simulink model "s_c107m32k_vlbi"  (R2018a)
settings: Solver=VariableStepDiscrete  StartTime=0.0  StopTime=(2^15)*10  RelTol=1e-3
undefined symbols (not defined in the file): fft_stages, n_bits_xengs
libraries: xbsIndex_r4 x23049, casper_library_misc x45, xps_library x4, casper_library_scopes x3, simulink x2
(part 41 of 201)

== system s_c107m32k_vlbi/DDC/dec_fir_async2 ==
  sync_in : Inport
  dv_in : Inport  Port=2
  real1 : Inport  Port=3
  imag1 : Inport  Port=4
  real2 : Inport  Port=5
  imag2 : Inport  Port=6
  real3 : Inport  Port=7
  imag3 : Inport  Port=8
  real4 : Inport  Port=9
  imag4 : Inport  Port=10
  real5 : Inport  Port=11
  imag5 : Inport  Port=12
  real6 : Inport  Port=13
  imag6 : Inport  Port=14
  real7 : Inport  Port=15
  imag7 : Inport  Port=16
  real8 : Inport  Port=17
  imag8 : Inport  Port=18
  real9 : Inport  Port=19
  imag9 : Inport  Port=20
  real10 : Inport  Port=21
  imag10 : Inport  Port=22
  real11 : Inport  Port=23
  imag11 : Inport  Port=24
  real12 : Inport  Port=25
  imag12 : Inport  Port=26
  real13 : Inport  Port=27
  imag13 : Inport  Port=28
  real14 : Inport  Port=29
  imag14 : Inport  Port=30
  real15 : Inport  Port=31
  imag15 : Inport  Port=32
  real16 : Inport  Port=33
  imag16 : Inport  Port=34
  convert1 : Subsystem  AncestorBlock=casper_library_misc/convert_of  mask(convert_of){bit_width_i=43, binary_point_i=34, bit_width_o=18, binary_point_o=17, csp_latency=7, overflow=Saturate, quantization=Round  (unbiased: even values)}
      mask prompts: bit_width_i "Bit Width In"; binary_point_i "Binary Point In"; bit_width_o "Bit Width Out"; binary_point_o "Binary Point Out"; csp_latency "Latency"; overflow "Overflow Behaviour"; quantization "Quantization Behaviour"
      mask help:
      | Converts from one 2's complement bit-width
      | and/or binary point position to another.
      | Includes underflow/overflow indicator.
      mask init: same as s_c107m32k_vlbi/DDC/bus_convert/conv1
      settings: AttributesFormatString=[43,34]->[18,17]
      mask TypeOptions overflow: Wrap | Saturate | Error
      mask TypeOptions quantization: Truncate | Round  (unbiased: +/- Inf) | Round  (unbiased: even values)
  convert2 : Subsystem  AncestorBlock=casper_library_misc/convert_of  mask(convert_of){bit_width_i=43, binary_point_i=34, bit_width_o=18, binary_point_o=17, csp_latency=7, overflow=Saturate, quantization=Round  (unbiased: even values)}
      mask prompts: bit_width_i "Bit Width In"; binary_point_i "Binary Point In"; bit_width_o "Bit Width Out"; binary_point_o "Binary Point Out"; csp_latency "Latency"; overflow "Overflow Behaviour"; quantization "Quantization Behaviour"
      mask help:
      | Converts from one 2's complement bit-width
      | and/or binary point position to another.
      | Includes underflow/overflow indicator.
      mask init: same as s_c107m32k_vlbi/DDC/bus_convert/conv1
      settings: AttributesFormatString=[43,34]->[18,17]
      mask TypeOptions overflow: Wrap | Saturate | Error
      mask TypeOptions quantization: Truncate | Round  (unbiased: +/- Inf) | Round  (unbiased: even values)
  dv_delay : xbsIndex_r4/Delay  rst=off  infoeditControl=Selection of Reset will increase slice count due to use of real FFs and instead of SRLs  en=off  latency=8  reg_retiming=off  dbl_ovrd=off  block_type=delay
  fir_col_async1 : Subsystem  AncestorBlock=casper_library_downconverter/fir_col_async  mask(fir_col_async){n_inputs=16, coeff=[-0.00014496 -9.1553e-05 -4.5776e-05 -7.6294e-06  2.2888e-05  4.5776e-05  6.1035e-05  7.6294e-05  7.6294e-05  7.6294e-05  7.6294e-05  6.8665e-05  6.1035e-05  5.3406e-05  4.5776e-05  8.3923e-05], add_latency=7, mult_latency=7, coeff_bit_width=18, coeff_bin_pt=17, first_stage_hdl=on, adder_imp=DSP48, async=on, bus_input=off, input_width=0, input_bp=0, input_type=Signed, dbl=on}
      mask prompts: n_inputs "Inputs"; coeff "Coefficients"; add_latency "Add latency"; mult_latency "Mult Latency"; coeff_bit_width "Coefficient bit width"; coeff_bin_pt "Coefficient binary point"; first_stage_hdl "Implement first stage of adder trees on output as behavioural HDL"; adder_imp "Adder implementation"; async "Asynchronous ops"; bus_input "Bus input"; input_width "Input bitwidth"; input_bp "Input binary point"; input_type "Input datatype"; dbl "Double col"
      mask init:
      | fir_col_async_init(gcb);
      mask Help: eval('xlWeb(''http://casper.berkeley.edu/wiki/Fir_col'')')
      mask TypeOptions adder_imp: Behavioral | Fabric | DSP48
      mask Callback bus_input:
      | onoff = get_param(gcb, 'bus_input');
      | set_param_state(gcb, 'input_width', onoff)
      | set_param_state(gcb, 'input_bp', onoff)
      | set_param_state(gcb, 'input_type', onoff)
      mask TypeOptions input_type: Signed | Unsigned
  fir_col_async2 : Subsystem  AncestorBlock=casper_library_downconverter/fir_col_async  mask(fir_col_async){n_inputs=16, coeff=[-0.00064087 -0.00073242 -0.00079346  -0.0008316 -0.00084686 -0.00083923 -0.00080872 -0.00077057 -0.00071716  -0.0006485 -0.00057983 -0.00050354 -0.00042725 -0.00035095 -0.00027466 -0.00021362], add_latency=7, mult_latency=7, coeff_bit_width=18, coeff_bin_pt=17, first_stage_hdl=on, adder_imp=DSP48, async=on, bus_input=off, input_width=0, input_bp=0, input_type=Signed, dbl=on}
      mask prompts: n_inputs "Inputs"; coeff "Coefficients"; add_latency "Add latency"; mult_latency "Mult Latency"; coeff_bit_width "Coefficient bit width"; coeff_bin_pt "Coefficient binary point"; first_stage_hdl "Implement first stage of adder trees on output as behavioural HDL"; adder_imp "Adder implementation"; async "Asynchronous ops"; bus_input "Bus input"; input_width "Input bitwidth"; input_bp "Input binary point"; input_type "Input datatype"; dbl "Double col"
      mask init:
      | fir_col_async_init(gcb);
      mask Help: eval('xlWeb(''http://casper.berkeley.edu/wiki/Fir_col'')')
      mask TypeOptions adder_imp: Behavioral | Fabric | DSP48
      mask Callback bus_input:
      | onoff = get_param(gcb, 'bus_input');
      | set_param_state(gcb, 'input_width', onoff)
      | set_param_state(gcb, 'input_bp', onoff)
      | set_param_state(gcb, 'input_type', onoff)
      mask TypeOptions input_type: Signed | Unsigned
  fir_col_async3 : Subsystem  AncestorBlock=casper_library_downconverter/fir_col_async  mask(fir_col_async){n_inputs=16, coeff=[0.0018005   0.0018311   0.0018005   0.0017242   0.0016022    0.001442   0.0012589   0.0010529   0.0008316  0.00061035  0.00038147  0.00016785 -3.8147e-05 -0.00022125 -0.00038147 -0.00052643], add_latency=7, mult_latency=7, coeff_bit_width=18, coeff_bin_pt=17, first_stage_hdl=on, adder_imp=DSP48, async=on, bus_input=off, input_width=0, input_bp=0, input_type=Signed, dbl=on}
      mask prompts: n_inputs "Inputs"; coeff "Coefficients"; add_latency "Add latency"; mult_latency "Mult Latency"; coeff_bit_width "Coefficient bit width"; coeff_bin_pt "Coefficient binary point"; first_stage_hdl "Implement first stage of adder trees on output as behavioural HDL"; adder_imp "Adder implementation"; async "Asynchronous ops"; bus_input "Bus input"; input_width "Input bitwidth"; input_bp "Input binary point"; input_type "Input datatype"; dbl "Double col"
      mask init:
      | fir_col_async_init(gcb);
      mask Help: eval('xlWeb(''http://casper.berkeley.edu/wiki/Fir_col'')')
      mask TypeOptions adder_imp: Behavioral | Fabric | DSP48
      mask Callback bus_input:
      | onoff = get_param(gcb, 'bus_input');
      | set_param_state(gcb, 'input_width', onoff)
      | set_param_state(gcb, 'input_bp', onoff)
      | set_param_state(gcb, 'input_type', onoff)
      mask TypeOptions input_type: Signed | Unsigned
  fir_col_async4 : Subsystem  AncestorBlock=casper_library_downconverter/fir_col_async  mask(fir_col_async){n_inputs=16, coeff=[-0.0036469  -0.0034409  -0.0031433  -0.0027847  -0.0023651  -0.0019073  -0.0014343 -0.00094604 -0.00047302 -2.2888e-05  0.00039673  0.00077057   0.0010986   0.0013657   0.0015717   0.0017166], add_latency=7, mult_latency=7, coeff_bit_width=18, coeff_bin_pt=17, first_stage_hdl=on, adder_imp=DSP48, async=on, bus_input=off, input_width=0, input_bp=0, input_type=Signed, dbl=on}
      mask prompts: n_inputs "Inputs"; coeff "Coefficients"; add_latency "Add latency"; mult_latency "Mult Latency"; coeff_bit_width "Coefficient bit width"; coeff_bin_pt "Coefficient binary point"; first_stage_hdl "Implement first stage of adder trees on output as behavioural HDL"; adder_imp "Adder implementation"; async "Asynchronous ops"; bus_input "Bus input"; input_width "Input bitwidth"; input_bp "Input binary point"; input_type "Input datatype"; dbl "Double col"
      mask init:
      | fir_col_async_init(gcb);
      mask Help: eval('xlWeb(''http://casper.berkeley.edu/wiki/Fir_col'')')
      mask TypeOptions adder_imp: Behavioral | Fabric | DSP48
      mask Callback bus_input:
      | onoff = get_param(gcb, 'bus_input');
      | set_param_state(gcb, 'input_width', onoff)
      | set_param_state(gcb, 'input_bp', onoff)
      | set_param_state(gcb, 'input_type', onoff)
      mask TypeOptions input_type: Signed | Unsigned
  fir_col_async5 : Subsystem  AncestorBlock=casper_library_downconverter/fir_col_async  mask(fir_col_async){n_inputs=16, coeff=[0.005806    0.005043   0.0041809   0.0032578   0.0023041   0.0013504  0.00042725 -0.00045013  -0.0012512  -0.0019608  -0.0025635  -0.0030518  -0.0034103  -0.0036469  -0.0037613  -0.0037613], add_latency=7, mult_latency=7, coeff_bit_width=18, coeff_bin_pt=17, first_stage_hdl=on, adder_imp=DSP48, async=on, bus_input=off, input_width=0, input_bp=0, input_type=Signed, dbl=on}
      mask prompts: n_inputs "Inputs"; coeff "Coefficients"; add_latency "Add latency"; mult_latency "Mult Latency"; coeff_bit_width "Coefficient bit width"; coeff_bin_pt "Coefficient binary point"; first_stage_hdl "Implement first stage of adder trees on output as behavioural HDL"; adder_imp "Adder implementation"; async "Asynchronous ops"; bus_input "Bus input"; input_width "Input bitwidth"; input_bp "Input binary point"; input_type "Input datatype"; dbl "Double col"
      mask init:
      | fir_col_async_init(gcb);
      mask Help: eval('xlWeb(''http://casper.berkeley.edu/wiki/Fir_col'')')
      mask TypeOptions adder_imp: Behavioral | Fabric | DSP48
      mask Callback bus_input:
      | onoff = get_param(gcb, 'bus_input');
      | set_param_state(gcb, 'input_width', onoff)
      | set_param_state(gcb, 'input_bp', onoff)
      | set_param_state(gcb, 'input_type', onoff)
      mask TypeOptions input_type: Signed | Unsigned
  fir_col_async6 : Subsystem  AncestorBlock=casper_library_downconverter/fir_col_async  mask(fir_col_async){n_inputs=16, coeff=[-0.007637  -0.0057373  -0.0038147  -0.0019302 -0.00013733   0.0015335   0.0030365   0.0043335   0.0054169   0.0062637   0.0068665    0.007225   0.0073471   0.0072403   0.0069351   0.0064468], add_latency=7, mult_latency=7, coeff_bit_width=18, coeff_bin_pt=17, first_stage_hdl=on, adder_imp=DSP48, async=on, bus_input=off, input_width=0, input_bp=0, input_type=Signed, dbl=on}
      mask prompts: n_inputs "Inputs"; coeff "Coefficients"; add_latency "Add latency"; mult_latency "Mult Latency"; coeff_bit_width "Coefficient bit width"; coeff_bin_pt "Coefficient binary point"; first_stage_hdl "Implement first stage of adder trees on output as behavioural HDL"; adder_imp "Adder implementation"; async "Asynchronous ops"; bus_input "Bus input"; input_width "Input bitwidth"; input_bp "Input binary point"; input_type "Input datatype"; dbl "Double col"
      mask init:
      | fir_col_async_init(gcb);
      mask Help: eval('xlWeb(''http://casper.berkeley.edu/wiki/Fir_col'')')
      mask TypeOptions adder_imp: Behavioral | Fabric | DSP48
      mask Callback bus_input:
      | onoff = get_param(gcb, 'bus_input');
      | set_param_state(gcb, 'input_width', onoff)
      | set_param_state(gcb, 'input_bp', onoff)
      | set_param_state(gcb, 'input_type', onoff)
      mask TypeOptions input_type: Signed | Unsigned
  fir_col_async7 : Subsystem  AncestorBlock=casper_library_downconverter/fir_col_async  mask(fir_col_async){n_inputs=16, coeff=[0.0078812   0.0032501 -0.00092316  -0.0046005  -0.0077515   -0.010345   -0.012383   -0.013863   -0.014809   -0.015228   -0.015175   -0.014679   -0.013809   -0.012604   -0.011131  -0.0094528], add_latency=7, mult_latency=7, coeff_bit_width=18, coeff_bin_pt=17, first_stage_hdl=on, adder_imp=DSP48, async=on, bus_input=off, input_width=0, input_bp=0, input_type=Signed, dbl=on}
      mask prompts: n_inputs "Inputs"; coeff "Coefficients"; add_latency "Add latency"; mult_latency "Mult Latency"; coeff_bit_width "Coefficient bit width"; coeff_bin_pt "Coefficient binary point"; first_stage_hdl "Implement first stage of adder trees on output as behavioural HDL"; adder_imp "Adder implementation"; async "Asynchronous ops"; bus_input "Bus input"; input_width "Input bitwidth"; input_bp "Input binary point"; input_type "Input datatype"; dbl "Double col"
      mask init:
      | fir_col_async_init(gcb);
      mask Help: eval('xlWeb(''http://casper.berkeley.edu/wiki/Fir_col'')')
      mask TypeOptions adder_imp: Behavioral | Fabric | DSP48
      mask Callback bus_input:
      | onoff = get_param(gcb, 'bus_input');
      | set_param_state(gcb, 'input_width', onoff)
      | set_param_state(gcb, 'input_bp', onoff)
      | set_param_state(gcb, 'input_type', onoff)
      mask TypeOptions input_type: Signed | Unsigned
  fir_col_async8 : Subsystem  AncestorBlock=casper_library_downconverter/fir_col_async  mask(fir_col_async){n_inputs=16, coeff=[0.077705     0.07692    0.075363    0.073059    0.070053    0.066406    0.062187    0.057465     0.05233    0.046883    0.041206    0.035408    0.029587    0.023834    0.018242    0.012901], add_latency=7, mult_latency=7, coeff_bit_width=18, coeff_bin_pt=17, first_stage_hdl=on, adder_imp=DSP48, async=on, bus_input=off, input_width=0, input_bp=0, input_type=Signed, dbl=on}
      mask prompts: n_inputs "Inputs"; coeff "Coefficients"; add_latency "Add latency"; mult_latency "Mult Latency"; coeff_bit_width "Coefficient bit width"; coeff_bin_pt "Coefficient binary point"; first_stage_hdl "Implement first stage of adder trees on output as behavioural HDL"; adder_imp "Adder implementation"; async "Asynchronous ops"; bus_input "Bus input"; input_width "Input bitwidth"; input_bp "Input binary point"; input_type "Input datatype"; dbl "Double col"
      mask init:
      | fir_col_async_init(gcb);
      mask Help: eval('xlWeb(''http://casper.berkeley.edu/wiki/Fir_col'')')
      mask TypeOptions adder_imp: Behavioral | Fabric | DSP48
      mask Callback bus_input:
      | onoff = get_param(gcb, 'bus_input');
      | set_param_state(gcb, 'input_width', onoff)
      | set_param_state(gcb, 'input_bp', onoff)
      | set_param_state(gcb, 'input_type', onoff)
      mask TypeOptions input_type: Signed | Unsigned
  imag_sum : Subsystem  AncestorBlock=casper_library_misc/adder_tree  mask(adder_tree){n_inputs=8, csp_latency=7, adder_imp=DSP48, first_stage_hdl=off, floating_point=off, dvalid_en=on, float_type=single, frac_width=0, exp_width=0}
      mask prompts: n_inputs "Number of Inputs"; csp_latency "Add Latency"; adder_imp "Adder implementation"; first_stage_hdl "Use behavioural HDL for first stage of adders"; floating_point "floating point"; float_type "float type"; frac_width "fraction length"; exp_width "exponent length"
      mask help:
      | Sums all inputs using a tree of adds and delays.
      |
      | Number of inputs: The number of inputs to the block to be summed
      | Add latency: The number of clock cycles to perform one addition (affects timing)..
      | Adder implementation: choice of fabric or DSP48E core, or behavioral HDL
      | Use behavioural HDL for first stage of adders: Causes the first stage of adders to be absorbed into DSP blocks if multipliers precede them (Virtex 5). Overrides Adder implementation
      mask init: same as s_c107m32k_vlbi/DDC/dec_fir_async/imag_sum
      settings: AttributesFormatString=latency 21
      mask Help: eval('xlWeb(''http://casper.berkeley.edu/wiki/Adder_tree'')')
      mask TypeOptions adder_imp: Behavioral | Fabric | DSP48
      mask Callback floating_point:
      | onoff = get_param(gcb, 'floating_point');
      | if strcmp(onoff,'on')
      |     enable_fixpt = 'off'
      |     set_param_state(gcb, 'float_type', 'on')
      | 
      |     f_type = get_param(gcb, 'float_type')
      |     if strcmp(f_type,'custom')
      |         set_param_state(gcb, 'exp_width', 'on')
      |         set_param_state(gcb, 'frac_width', 'on')
      |     else
      |         set_param_state(gcb, 'exp_width', 'off')
      |         set_param_state(gcb, 'frac_width', 'off')
      |     end
      | 
      | 
      | else
      |     enable_fixpt = 'on'
      |     set_param_state(gcb, 'float_type', 'off')
      |     set_param_state(gcb, 'exp_width', 'off')
      |     set_param_state(gcb, 'frac_width', 'off')
      | end
      mask TypeOptions float_type: single | custom
      mask Callback float_type:
      | f_type = get_param(gcb, 'float_type')
      | if strcmp(f_type,'custom')
      |     set_param_state(gcb, 'exp_width', 'on')
      |     set_param_state(gcb, 'frac_width', 'on')
      | else
      |     set_param_state(gcb, 'exp_width', 'off')
      |     set_param_state(gcb, 'frac_width', 'off')
      | end
  or_reduce : xbsIndex_r4/Logical  logical_function=OR  inputs=2  en=off  latency=1  precision=Full  arith_type=Unsigned  n_bits=16  bin_pt=0  align_bp=on  dbl_ovrd=off  block_type=logical
  real_sum : Subsystem  AncestorBlock=casper_library_misc/adder_tree  mask(adder_tree){n_inputs=8, csp_latency=7, adder_imp=DSP48, first_stage_hdl=off, floating_point=off, dvalid_en=on, float_type=single, frac_width=0, exp_width=0}
      mask prompts: n_inputs "Number of Inputs"; csp_latency "Add Latency"; adder_imp "Adder implementation"; first_stage_hdl "Use behavioural HDL for first stage of adders"; floating_point "floating point"; float_type "float type"; frac_width "fraction length"; exp_width "exponent length"
      mask help:
      | Sums all inputs using a tree of adds and delays.
      |
      | Number of inputs: The number of inputs to the block to be summed
      | Add latency: The number of clock cycles to perform one addition (affects timing)..
      | Adder implementation: choice of fabric or DSP48E core, or behavioral HDL
      | Use behavioural HDL for first stage of adders: Causes the first stage of adders to be absorbed into DSP blocks if multipliers precede them (Virtex 5). Overrides Adder implementation
      mask init: same as s_c107m32k_vlbi/DDC/dec_fir_async/imag_sum
      settings: AttributesFormatString=latency 21
      mask Help: eval('xlWeb(''http://casper.berkeley.edu/wiki/Adder_tree'')')
      mask TypeOptions adder_imp: Behavioral | Fabric | DSP48
      mask Callback floating_point:
      | onoff = get_param(gcb, 'floating_point');
      | if strcmp(onoff,'on')
      |     enable_fixpt = 'off'
      |     set_param_state(gcb, 'float_type', 'on')
      | 
      |     f_type = get_param(gcb, 'float_type')
      |     if strcmp(f_type,'custom')
      |         set_param_state(gcb, 'exp_width', 'on')
      |         set_param_state(gcb, 'frac_width', 'on')
      |     else
      |         set_param_state(gcb, 'exp_width', 'off')
      |         set_param_state(gcb, 'frac_width', 'off')
      |     end
      | 
      | 
      | else
      |     enable_fixpt = 'on'
      |     set_param_state(gcb, 'float_type', 'off')
      |     set_param_state(gcb, 'exp_width', 'off')
      |     set_param_state(gcb, 'frac_width', 'off')
      | end
      mask TypeOptions float_type: single | custom
      mask Callback float_type:
      | f_type = get_param(gcb, 'float_type')
      | if strcmp(f_type,'custom')
      |     set_param_state(gcb, 'exp_width', 'on')
      |     set_param_state(gcb, 'frac_width', 'on')
      | else
      |     set_param_state(gcb, 'exp_width', 'off')
      |     set_param_state(gcb, 'frac_width', 'off')
      | end
  ri_to_c : casper_library_misc/ri_to_c
      settings: SourceProductName=CASPER DSP Blockset
  shift1 : xbsIndex_r4/Shift  shift_dir=Left  shift_bits=0  en=off  latency=1  precision=Full  arith_type="Signed  (2's comp)"  n_bits=16  bin_pt=14  quantization=Truncate  overflow=Wrap  dbl_ovrd=off  block_type=shift
  shift2 : xbsIndex_r4/Shift  shift_dir=Left  shift_bits=0  en=off  latency=1  precision=Full  arith_type="Signed  (2's comp)"  n_bits=16  bin_pt=14  quantization=Truncate  overflow=Wrap  dbl_ovrd=off  block_type=shift
  sync_delay : xbsIndex_r4/Delay  rst=off  infoeditControl=Selection of Reset will increase slice count due to use of real FFs and instead of SRLs  en=on  latency=49  reg_retiming=off  dbl_ovrd=off  block_type=delay
  sync_out : Outport
  dout : Outport  Port=2
  of_out : Outport  Port=3
  dv_out : Outport  Port=4
  wires:
  sync_in/1 -> sync_delay/1
  dv_in/1 -> dv_delay/1, sync_delay/2, fir_col_async1/65(dv), fir_col_async2/65(dv), fir_col_async3/65(dv), fir_col_async4/65(dv), fir_col_async5/65(dv), fir_col_async6/65(dv), fir_col_async7/65(dv), fir_col_async8/65(dv), real_sum/1(dv_in), imag_sum/1(dv_in)
  dv_delay/1 -> dv_out/1
  real1/1 -> fir_col_async1/1(real1)
  imag1/1 -> fir_col_async1/2(imag1)
  real2/1 -> fir_col_async1/3(real2)
  imag2/1 -> fir_col_async1/4(imag2)
  real3/1 -> fir_col_async1/5(real3)
  imag3/1 -> fir_col_async1/6(imag3)
  real4/1 -> fir_col_async1/7(real4)
  imag4/1 -> fir_col_async1/8(imag4)
  real5/1 -> fir_col_async1/9(real5)
  imag5/1 -> fir_col_async1/10(imag5)
  real6/1 -> fir_col_async1/11(real6)
  imag6/1 -> fir_col_async1/12(imag6)
  real7/1 -> fir_col_async1/13(real7)
  imag7/1 -> fir_col_async1/14(imag7)
  real8/1 -> fir_col_async1/15(real8)
  imag8/1 -> fir_col_async1/16(imag8)
  real9/1 -> fir_col_async1/17(real9)
  imag9/1 -> fir_col_async1/18(imag9)
  real10/1 -> fir_col_async1/19(real10)
  imag10/1 -> fir_col_async1/20(imag10)
  real11/1 -> fir_col_async1/21(real11)
  imag11/1 -> fir_col_async1/22(imag11)
  real12/1 -> fir_col_async1/23(real12)
  imag12/1 -> fir_col_async1/24(imag12)
  real13/1 -> fir_col_async1/25(real13)
  imag13/1 -> fir_col_async1/26(imag13)
  real14/1 -> fir_col_async1/27(real14)
  imag14/1 -> fir_col_async1/28(imag14)
  real15/1 -> fir_col_async1/29(real15)
  imag15/1 -> fir_col_async1/30(imag15)
  real16/1 -> fir_col_async1/31(real16)
  imag16/1 -> fir_col_async1/32(imag16)
  fir_col_async1/65(real_sum) -> real_sum/3(din1)
  fir_col_async1/66(imag_sum) -> imag_sum/3(din1)
  fir_col_async1/1(real_out1) -> fir_col_async2/1(real1)
  fir_col_async1/2(imag_out1) -> fir_col_async2/2(imag1)
  fir_col_async1/3(real_out2) -> fir_col_async2/3(real2)
  fir_col_async1/4(imag_out2) -> fir_col_async2/4(imag2)
  fir_col_async1/5(real_out3) -> fir_col_async2/5(real3)
  fir_col_async1/6(imag_out3) -> fir_col_async2/6(imag3)
  fir_col_async1/7(real_out4) -> fir_col_async2/7(real4)
  fir_col_async1/8(imag_out4) -> fir_col_async2/8(imag4)
  fir_col_async1/9(real_out5) -> fir_col_async2/9(real5)
  fir_col_async1/10(imag_out5) -> fir_col_async2/10(imag5)
  fir_col_async1/11(real_out6) -> fir_col_async2/11(real6)
  fir_col_async1/12(imag_out6) -> fir_col_async2/12(imag6)
  fir_col_async1/13(real_out7) -> fir_col_async2/13(real7)
  fir_col_async1/14(imag_out7) -> fir_col_async2/14(imag7)
  fir_col_async1/15(real_out8) -> fir_col_async2/15(real8)
  fir_col_async1/16(imag_out8) -> fir_col_async2/16(imag8)
  fir_col_async1/17(real_out9) -> fir_col_async2/17(real9)
  fir_col_async1/18(imag_out9) -> fir_col_async2/18(imag9)
  fir_col_async1/19(real_out10) -> fir_col_async2/19(real10)
  fir_col_async1/20(imag_out10) -> fir_col_async2/20(imag10)
  fir_col_async1/21(real_out11) -> fir_col_async2/21(real11)
  fir_col_async1/22(imag_out11) -> fir_col_async2/22(imag11)
  fir_col_async1/23(real_out12) -> fir_col_async2/23(real12)
  fir_col_async1/24(imag_out12) -> fir_col_async2/24(imag12)
  fir_col_async1/25(real_out13) -> fir_col_async2/25(real13)
  fir_col_async1/26(imag_out13) -> fir_col_async2/26(imag13)
  fir_col_async1/27(real_out14) -> fir_col_async2/27(real14)
  fir_col_async1/28(imag_out14) -> fir_col_async2/28(imag14)
  fir_col_async1/29(real_out15) -> fir_col_async2/29(real15)
  fir_col_async1/30(imag_out15) -> fir_col_async2/30(imag15)
  fir_col_async1/31(real_out16) -> fir_col_async2/31(real16)
  fir_col_async1/32(imag_out16) -> fir_col_async2/32(imag16)
  fir_col_async2/65(real_sum) -> real_sum/4(din2)
  fir_col_async2/66(imag_sum) -> imag_sum/4(din2)
  fir_col_async2/1(real_out1) -> fir_col_async3/1(real1)
  fir_col_async2/2(imag_out1) -> fir_col_async3/2(imag1)
  fir_col_async2/3(real_out2) -> fir_col_async3/3(real2)
  fir_col_async2/4(imag_out2) -> fir_col_async3/4(imag2)
  fir_col_async2/5(real_out3) -> fir_col_async3/5(real3)
  fir_col_async2/6(imag_out3) -> fir_col_async3/6(imag3)
  fir_col_async2/7(real_out4) -> fir_col_async3/7(real4)
  fir_col_async2/8(imag_out4) -> fir_col_async3/8(imag4)
  fir_col_async2/9(real_out5) -> fir_col_async3/9(real5)
  fir_col_async2/10(imag_out5) -> fir_col_async3/10(imag5)
  fir_col_async2/11(real_out6) -> fir_col_async3/11(real6)
  fir_col_async2/12(imag_out6) -> fir_col_async3/12(imag6)
  fir_col_async2/13(real_out7) -> fir_col_async3/13(real7)
  fir_col_async2/14(imag_out7) -> fir_col_async3/14(imag7)
  fir_col_async2/15(real_out8) -> fir_col_async3/15(real8)
  fir_col_async2/16(imag_out8) -> fir_col_async3/16(imag8)
  fir_col_async2/17(real_out9) -> fir_col_async3/17(real9)
  fir_col_async2/18(imag_out9) -> fir_col_async3/18(imag9)
  fir_col_async2/19(real_out10) -> fir_col_async3/19(real10)
  fir_col_async2/20(imag_out10) -> fir_col_async3/20(imag10)
  fir_col_async2/21(real_out11) -> fir_col_async3/21(real11)
  fir_col_async2/22(imag_out11) -> fir_col_async3/22(imag11)
  fir_col_async2/23(real_out12) -> fir_col_async3/23(real12)
  fir_col_async2/24(imag_out12) -> fir_col_async3/24(imag12)
  fir_col_async2/25(real_out13) -> fir_col_async3/25(real13)
  fir_col_async2/26(imag_out13) -> fir_col_async3/26(imag13)
  fir_col_async2/27(real_out14) -> fir_col_async3/27(real14)
  fir_col_async2/28(imag_out14) -> fir_col_async3/28(imag14)
  fir_col_async2/29(real_out15) -> fir_col_async3/29(real15)
  fir_col_async2/30(imag_out15) -> fir_col_async3/30(imag15)
  fir_col_async2/31(real_out16) -> fir_col_async3/31(real16)
  fir_col_async2/32(imag_out16) -> fir_col_async3/32(imag16)
  fir_col_async3/65(real_sum) -> real_sum/5(din3)
  fir_col_async3/66(imag_sum) -> imag_sum/5(din3)
  fir_col_async3/1(real_out1) -> fir_col_async4/1(real1)
  fir_col_async3/2(imag_out1) -> fir_col_async4/2(imag1)
  fir_col_async3/3(real_out2) -> fir_col_async4/3(real2)
  fir_col_async3/4(imag_out2) -> fir_col_async4/4(imag2)
  fir_col_async3/5(real_out3) -> fir_col_async4/5(real3)
  fir_col_async3/6(imag_out3) -> fir_col_async4/6(imag3)
  fir_col_async3/7(real_out4) -> fir_col_async4/7(real4)
  fir_col_async3/8(imag_out4) -> fir_col_async4/8(imag4)
  fir_col_async3/9(real_out5) -> fir_col_async4/9(real5)
  fir_col_async3/10(imag_out5) -> fir_col_async4/10(imag5)
  fir_col_async3/11(real_out6) -> fir_col_async4/11(real6)
  fir_col_async3/12(imag_out6) -> fir_col_async4/12(imag6)
  fir_col_async3/13(real_out7) -> fir_col_async4/13(real7)
  fir_col_async3/14(imag_out7) -> fir_col_async4/14(imag7)
  fir_col_async3/15(real_out8) -> fir_col_async4/15(real8)
  fir_col_async3/16(imag_out8) -> fir_col_async4/16(imag8)
  fir_col_async3/17(real_out9) -> fir_col_async4/17(real9)
  fir_col_async3/18(imag_out9) -> fir_col_async4/18(imag9)
  fir_col_async3/19(real_out10) -> fir_col_async4/19(real10)
  fir_col_async3/20(imag_out10) -> fir_col_async4/20(imag10)
  fir_col_async3/21(real_out11) -> fir_col_async4/21(real11)
  fir_col_async3/22(imag_out11) -> fir_col_async4/22(imag11)
  fir_col_async3/23(real_out12) -> fir_col_async4/23(real12)
  fir_col_async3/24(imag_out12) -> fir_col_async4/24(imag12)
  fir_col_async3/25(real_out13) -> fir_col_async4/25(real13)
  fir_col_async3/26(imag_out13) -> fir_col_async4/26(imag13)
  fir_col_async3/27(real_out14) -> fir_col_async4/27(real14)
  fir_col_async3/28(imag_out14) -> fir_col_async4/28(imag14)
  fir_col_async3/29(real_out15) -> fir_col_async4/29(real15)
  fir_col_async3/30(imag_out15) -> fir_col_async4/30(imag15)
  fir_col_async3/31(real_out16) -> fir_col_async4/31(real16)
  fir_col_async3/32(imag_out16) -> fir_col_async4/32(imag16)
  fir_col_async4/65(real_sum) -> real_sum/6(din4)
  fir_col_async4/66(imag_sum) -> imag_sum/6(din4)
  fir_col_async4/1(real_out1) -> fir_col_async5/1(real1)
  fir_col_async4/2(imag_out1) -> fir_col_async5/2(imag1)
  fir_col_async4/3(real_out2) -> fir_col_async5/3(real2)
  fir_col_async4/4(imag_out2) -> fir_col_async5/4(imag2)
  fir_col_async4/5(real_out3) -> fir_col_async5/5(real3)
  fir_col_async4/6(imag_out3) -> fir_col_async5/6(imag3)
  fir_col_async4/7(real_out4) -> fir_col_async5/7(real4)
  fir_col_async4/8(imag_out4) -> fir_col_async5/8(imag4)
  fir_col_async4/9(real_out5) -> fir_col_async5/9(real5)
  fir_col_async4/10(imag_out5) -> fir_col_async5/10(imag5)
  fir_col_async4/11(real_out6) -> fir_col_async5/11(real6)
  fir_col_async4/12(imag_out6) -> fir_col_async5/12(imag6)
  fir_col_async4/13(real_out7) -> fir_col_async5/13(real7)
  fir_col_async4/14(imag_out7) -> fir_col_async5/14(imag7)
  fir_col_async4/15(real_out8) -> fir_col_async5/15(real8)
  fir_col_async4/16(imag_out8) -> fir_col_async5/16(imag8)
  fir_col_async4/17(real_out9) -> fir_col_async5/17(real9)
  fir_col_async4/18(imag_out9) -> fir_col_async5/18(imag9)
  fir_col_async4/19(real_out10) -> fir_col_async5/19(real10)
  fir_col_async4/20(imag_out10) -> fir_col_async5/20(imag10)
  fir_col_async4/21(real_out11) -> fir_col_async5/21(real11)
  fir_col_async4/22(imag_out11) -> fir_col_async5/22(imag11)
  fir_col_async4/23(real_out12) -> fir_col_async5/23(real12)
  fir_col_async4/24(imag_out12) -> fir_col_async5/24(imag12)
  fir_col_async4/25(real_out13) -> fir_col_async5/25(real13)
  fir_col_async4/26(imag_out13) -> fir_col_async5/26(imag13)
  fir_col_async4/27(real_out14) -> fir_col_async5/27(real14)
  fir_col_async4/28(imag_out14) -> fir_col_async5/28(imag14)
  fir_col_async4/29(real_out15) -> fir_col_async5/29(real15)
  fir_col_async4/30(imag_out15) -> fir_col_async5/30(imag15)
  fir_col_async4/31(real_out16) -> fir_col_async5/31(real16)
  fir_col_async4/32(imag_out16) -> fir_col_async5/32(imag16)
  fir_col_async5/65(real_sum) -> real_sum/7(din5)
  fir_col_async5/66(imag_sum) -> imag_sum/7(din5)
  fir_col_async5/1(real_out1) -> fir_col_async6/1(real1)
  fir_col_async5/2(imag_out1) -> fir_col_async6/2(imag1)
  fir_col_async5/3(real_out2) -> fir_col_async6/3(real2)
  fir_col_async5/4(imag_out2) -> fir_col_async6/4(imag2)
  fir_col_async5/5(real_out3) -> fir_col_async6/5(real3)
  fir_col_async5/6(imag_out3) -> fir_col_async6/6(imag3)
  fir_col_async5/7(real_out4) -> fir_col_async6/7(real4)
  fir_col_async5/8(imag_out4) -> fir_col_async6/8(imag4)
  fir_col_async5/9(real_out5) -> fir_col_async6/9(real5)
  fir_col_async5/10(imag_out5) -> fir_col_async6/10(imag5)
  fir_col_async5/11(real_out6) -> fir_col_async6/11(real6)
  fir_col_async5/12(imag_out6) -> fir_col_async6/12(imag6)
  fir_col_async5/13(real_out7) -> fir_col_async6/13(real7)
  fir_col_async5/14(imag_out7) -> fir_col_async6/14(imag7)
  fir_col_async5/15(real_out8) -> fir_col_async6/15(real8)
  fir_col_async5/16(imag_out8) -> fir_col_async6/16(imag8)
  fir_col_async5/17(real_out9) -> fir_col_async6/17(real9)
  fir_col_async5/18(imag_out9) -> fir_col_async6/18(imag9)
  fir_col_async5/19(real_out10) -> fir_col_async6/19(real10)
  fir_col_async5/20(imag_out10) -> fir_col_async6/20(imag10)
  fir_col_async5/21(real_out11) -> fir_col_async6/21(real11)
  fir_col_async5/22(imag_out11) -> fir_col_async6/22(imag11)
  fir_col_async5/23(real_out12) -> fir_col_async6/23(real12)
  fir_col_async5/24(imag_out12) -> fir_col_async6/24(imag12)
  fir_col_async5/25(real_out13) -> fir_col_async6/25(real13)
  fir_col_async5/26(imag_out13) -> fir_col_async6/26(imag13)
  fir_col_async5/27(real_out14) -> fir_col_async6/27(real14)
  fir_col_async5/28(imag_out14) -> fir_col_async6/28(imag14)
  fir_col_async5/29(real_out15) -> fir_col_async6/29(real15)
  fir_col_async5/30(imag_out15) -> fir_col_async6/30(imag15)
  fir_col_async5/31(real_out16) -> fir_col_async6/31(real16)
  fir_col_async5/32(imag_out16) -> fir_col_async6/32(imag16)
  fir_col_async6/65(real_sum) -> real_sum/8(din6)
  fir_col_async6/66(imag_sum) -> imag_sum/8(din6)
  fir_col_async6/1(real_out1) -> fir_col_async7/1(real1)
  fir_col_async6/2(imag_out1) -> fir_col_async7/2(imag1)
  fir_col_async6/3(real_out2) -> fir_col_async7/3(real2)
  fir_col_async6/4(imag_out2) -> fir_col_async7/4(imag2)
  fir_col_async6/5(real_out3) -> fir_col_async7/5(real3)
  fir_col_async6/6(imag_out3) -> fir_col_async7/6(imag3)
  fir_col_async6/7(real_out4) -> fir_col_async7/7(real4)
  fir_col_async6/8(imag_out4) -> fir_col_async7/8(imag4)
  fir_col_async6/9(real_out5) -> fir_col_async7/9(real5)
  fir_col_async6/10(imag_out5) -> fir_col_async7/10(imag5)
  fir_col_async6/11(real_out6) -> fir_col_async7/11(real6)
  fir_col_async6/12(imag_out6) -> fir_col_async7/12(imag6)
  fir_col_async6/13(real_out7) -> fir_col_async7/13(real7)
  fir_col_async6/14(imag_out7) -> fir_col_async7/14(imag7)
  fir_col_async6/15(real_out8) -> fir_col_async7/15(real8)
  fir_col_async6/16(imag_out8) -> fir_col_async7/16(imag8)
  fir_col_async6/17(real_out9) -> fir_col_async7/17(real9)
  fir_col_async6/18(imag_out9) -> fir_col_async7/18(imag9)
  fir_col_async6/19(real_out10) -> fir_col_async7/19(real10)
  fir_col_async6/20(imag_out10) -> fir_col_async7/20(imag10)
  fir_col_async6/21(real_out11) -> fir_col_async7/21(real11)
  fir_col_async6/22(imag_out11) -> fir_col_async7/22(imag11)
  fir_col_async6/23(real_out12) -> fir_col_async7/23(real12)
  fir_col_async6/24(imag_out12) -> fir_col_async7/24(imag12)
  fir_col_async6/25(real_out13) -> fir_col_async7/25(real13)
  fir_col_async6/26(imag_out13) -> fir_col_async7/26(imag13)
  fir_col_async6/27(real_out14) -> fir_col_async7/27(real14)
  fir_col_async6/28(imag_out14) -> fir_col_async7/28(imag14)
  fir_col_async6/29(real_out15) -> fir_col_async7/29(real15)
  fir_col_async6/30(imag_out15) -> fir_col_async7/30(imag15)
  fir_col_async6/31(real_out16) -> fir_col_async7/31(real16)
  fir_col_async6/32(imag_out16) -> fir_col_async7/32(imag16)
  fir_col_async7/65(real_sum) -> real_sum/9(din7)
  fir_col_async7/66(imag_sum) -> imag_sum/9(din7)
  fir_col_async7/1(real_out1) -> fir_col_async8/1(real1)
  fir_col_async7/2(imag_out1) -> fir_col_async8/2(imag1)
  fir_col_async7/3(real_out2) -> fir_col_async8/3(real2)
  fir_col_async7/4(imag_out2) -> fir_col_async8/4(imag2)
  fir_col_async7/5(real_out3) -> fir_col_async8/5(real3)
  fir_col_async7/6(imag_out3) -> fir_col_async8/6(imag3)
  fir_col_async7/7(real_out4) -> fir_col_async8/7(real4)
  fir_col_async7/8(imag_out4) -> fir_col_async8/8(imag4)
  fir_col_async7/9(real_out5) -> fir_col_async8/9(real5)
  fir_col_async7/10(imag_out5) -> fir_col_async8/10(imag5)
  fir_col_async7/11(real_out6) -> fir_col_async8/11(real6)
  fir_col_async7/12(imag_out6) -> fir_col_async8/12(imag6)
  fir_col_async7/13(real_out7) -> fir_col_async8/13(real7)
  fir_col_async7/14(imag_out7) -> fir_col_async8/14(imag7)
  fir_col_async7/15(real_out8) -> fir_col_async8/15(real8)
  fir_col_async7/16(imag_out8) -> fir_col_async8/16(imag8)
  fir_col_async7/17(real_out9) -> fir_col_async8/17(real9)
  fir_col_async7/18(imag_out9) -> fir_col_async8/18(imag9)
  fir_col_async7/19(real_out10) -> fir_col_async8/19(real10)
  fir_col_async7/20(imag_out10) -> fir_col_async8/20(imag10)
  fir_col_async7/21(real_out11) -> fir_col_async8/21(real11)
  fir_col_async7/22(imag_out11) -> fir_col_async8/22(imag11)
  fir_col_async7/23(real_out12) -> fir_col_async8/23(real12)
  fir_col_async7/24(imag_out12) -> fir_col_async8/24(imag12)
  fir_col_async7/25(real_out13) -> fir_col_async8/25(real13)
  fir_col_async7/26(imag_out13) -> fir_col_async8/26(imag13)
  fir_col_async7/27(real_out14) -> fir_col_async8/27(real14)
  fir_col_async7/28(imag_out14) -> fir_col_async8/28(imag14)
  fir_col_async7/29(real_out15) -> fir_col_async8/29(real15)
  fir_col_async7/30(imag_out15) -> fir_col_async8/30(imag15)
  fir_col_async7/31(real_out16) -> fir_col_async8/31(real16)
  fir_col_async7/32(imag_out16) -> fir_col_async8/32(imag16)
  fir_col_async8/65(real_sum) -> real_sum/10(din8)
  fir_col_async8/66(imag_sum) -> imag_sum/10(din8)
  real_sum/2(dout) -> shift1/1
  imag_sum/2(dout) -> shift2/1
  shift1/1 -> convert1/1(din)
  shift2/1 -> convert2/1(din)
  convert1/1(dout) -> ri_to_c/1
  convert1/2(of) -> or_reduce/1
  convert2/1(dout) -> ri_to_c/2
  convert2/2(of) -> or_reduce/2
  or_reduce/1 -> of_out/1
  ri_to_c/1 -> dout/1
  real_sum/1(sync_out) -> sync_out/1
  sync_delay/1 -> real_sum/2(sync), imag_sum/2(sync)
  fir_col_async2/33(real_back_out1) -> fir_col_async1/33(real_back1)
  fir_col_async2/34(imag_back_out1) -> fir_col_async1/34(imag_back1)
  fir_col_async2/35(real_back_out2) -> fir_col_async1/35(real_back2)
  fir_col_async2/36(imag_back_out2) -> fir_col_async1/36(imag_back2)
  fir_col_async2/37(real_back_out3) -> fir_col_async1/37(real_back3)
  fir_col_async2/38(imag_back_out3) -> fir_col_async1/38(imag_back3)
  fir_col_async2/39(real_back_out4) -> fir_col_async1/39(real_back4)
  fir_col_async2/40(imag_back_out4) -> fir_col_async1/40(imag_back4)
  fir_col_async2/41(real_back_out5) -> fir_col_async1/41(real_back5)
  fir_col_async2/42(imag_back_out5) -> fir_col_async1/42(imag_back5)
  fir_col_async2/43(real_back_out6) -> fir_col_async1/43(real_back6)
  fir_col_async2/44(imag_back_out6) -> fir_col_async1/44(imag_back6)
  fir_col_async2/45(real_back_out7) -> fir_col_async1/45(real_back7)
  fir_col_async2/46(imag_back_out7) -> fir_col_async1/46(imag_back7)
  fir_col_async2/47(real_back_out8) -> fir_col_async1/47(real_back8)
  fir_col_async2/48(imag_back_out8) -> fir_col_async1/48(imag_back8)
  fir_col_async2/49(real_back_out9) -> fir_col_async1/49(real_back9)
  fir_col_async2/50(imag_back_out9) -> fir_col_async1/50(imag_back9)
  fir_col_async2/51(real_back_out10) -> fir_col_async1/51(real_back10)
  fir_col_async2/52(imag_back_out10) -> fir_col_async1/52(imag_back10)
  fir_col_async2/53(real_back_out11) -> fir_col_async1/53(real_back11)
  fir_col_async2/54(imag_back_out11) -> fir_col_async1/54(imag_back11)
  fir_col_async2/55(real_back_out12) -> fir_col_async1/55(real_back12)
  fir_col_async2/56(imag_back_out12) -> fir_col_async1/56(imag_back12)
  fir_col_async2/57(real_back_out13) -> fir_col_async1/57(real_back13)
  fir_col_async2/58(imag_back_out13) -> fir_col_async1/58(imag_back13)
  fir_col_async2/59(real_back_out14) -> fir_col_async1/59(real_back14)
  fir_col_async2/60(imag_back_out14) -> fir_col_async1/60(imag_back14)
  fir_col_async2/61(real_back_out15) -> fir_col_async1/61(real_back15)
  fir_col_async2/62(imag_back_out15) -> fir_col_async1/62(imag_back15)
  fir_col_async2/63(real_back_out16) -> fir_col_async1/63(real_back16)
  fir_col_async2/64(imag_back_out16) -> fir_col_async1/64(imag_back16)
  fir_col_async3/33(real_back_out1) -> fir_col_async2/33(real_back1)
  fir_col_async3/34(imag_back_out1) -> fir_col_async2/34(imag_back1)
  fir_col_async3/35(real_back_out2) -> fir_col_async2/35(real_back2)
  fir_col_async3/36(imag_back_out2) -> fir_col_async2/36(imag_back2)
  fir_col_async3/37(real_back_out3) -> fir_col_async2/37(real_back3)
  fir_col_async3/38(imag_back_out3) -> fir_col_async2/38(imag_back3)
  fir_col_async3/39(real_back_out4) -> fir_col_async2/39(real_back4)
  fir_col_async3/40(imag_back_out4) -> fir_col_async2/40(imag_back4)
  fir_col_async3/41(real_back_out5) -> fir_col_async2/41(real_back5)
  fir_col_async3/42(imag_back_out5) -> fir_col_async2/42(imag_back5)
  fir_col_async3/43(real_back_out6) -> fir_col_async2/43(real_back6)
  fir_col_async3/44(imag_back_out6) -> fir_col_async2/44(imag_back6)
  fir_col_async3/45(real_back_out7) -> fir_col_async2/45(real_back7)
  fir_col_async3/46(imag_back_out7) -> fir_col_async2/46(imag_back7)
  fir_col_async3/47(real_back_out8) -> fir_col_async2/47(real_back8)
  fir_col_async3/48(imag_back_out8) -> fir_col_async2/48(imag_back8)
  fir_col_async3/49(real_back_out9) -> fir_col_async2/49(real_back9)
  fir_col_async3/50(imag_back_out9) -> fir_col_async2/50(imag_back9)
  fir_col_async3/51(real_back_out10) -> fir_col_async2/51(real_back10)
  fir_col_async3/52(imag_back_out10) -> fir_col_async2/52(imag_back10)
  fir_col_async3/53(real_back_out11) -> fir_col_async2/53(real_back11)
  fir_col_async3/54(imag_back_out11) -> fir_col_async2/54(imag_back11)
  fir_col_async3/55(real_back_out12) -> fir_col_async2/55(real_back12)
  fir_col_async3/56(imag_back_out12) -> fir_col_async2/56(imag_back12)
  fir_col_async3/57(real_back_out13) -> fir_col_async2/57(real_back13)
  fir_col_async3/58(imag_back_out13) -> fir_col_async2/58(imag_back13)
  fir_col_async3/59(real_back_out14) -> fir_col_async2/59(real_back14)
  fir_col_async3/60(imag_back_out14) -> fir_col_async2/60(imag_back14)
  fir_col_async3/61(real_back_out15) -> fir_col_async2/61(real_back15)
  fir_col_async3/62(imag_back_out15) -> fir_col_async2/62(imag_back15)
  fir_col_async3/63(real_back_out16) -> fir_col_async2/63(real_back16)
  fir_col_async3/64(imag_back_out16) -> fir_col_async2/64(imag_back16)
  fir_col_async4/33(real_back_out1) -> fir_col_async3/33(real_back1)
  fir_col_async4/34(imag_back_out1) -> fir_col_async3/34(imag_back1)
  fir_col_async4/35(real_back_out2) -> fir_col_async3/35(real_back2)
  fir_col_async4/36(imag_back_out2) -> fir_col_async3/36(imag_back2)
  fir_col_async4/37(real_back_out3) -> fir_col_async3/37(real_back3)
  fir_col_async4/38(imag_back_out3) -> fir_col_async3/38(imag_back3)
  fir_col_async4/39(real_back_out4) -> fir_col_async3/39(real_back4)
  fir_col_async4/40(imag_back_out4) -> fir_col_async3/40(imag_back4)
  fir_col_async4/41(real_back_out5) -> fir_col_async3/41(real_back5)
  fir_col_async4/42(imag_back_out5) -> fir_col_async3/42(imag_back5)
  fir_col_async4/43(real_back_out6) -> fir_col_async3/43(real_back6)
  fir_col_async4/44(imag_back_out6) -> fir_col_async3/44(imag_back6)
  fir_col_async4/45(real_back_out7) -> fir_col_async3/45(real_back7)
  fir_col_async4/46(imag_back_out7) -> fir_col_async3/46(imag_back7)
  fir_col_async4/47(real_back_out8) -> fir_col_async3/47(real_back8)
  fir_col_async4/48(imag_back_out8) -> fir_col_async3/48(imag_back8)
  fir_col_async4/49(real_back_out9) -> fir_col_async3/49(real_back9)
  fir_col_async4/50(imag_back_out9) -> fir_col_async3/50(imag_back9)
  fir_col_async4/51(real_back_out10) -> fir_col_async3/51(real_back10)
  fir_col_async4/52(imag_back_out10) -> fir_col_async3/52(imag_back10)
  fir_col_async4/53(real_back_out11) -> fir_col_async3/53(real_back11)
  fir_col_async4/54(imag_back_out11) -> fir_col_async3/54(imag_back11)
  fir_col_async4/55(real_back_out12) -> fir_col_async3/55(real_back12)
  fir_col_async4/56(imag_back_out12) -> fir_col_async3/56(imag_back12)
  fir_col_async4/57(real_back_out13) -> fir_col_async3/57(real_back13)
  fir_col_async4/58(imag_back_out13) -> fir_col_async3/58(imag_back13)
  fir_col_async4/59(real_back_out14) -> fir_col_async3/59(real_back14)
  fir_col_async4/60(imag_back_out14) -> fir_col_async3/60(imag_back14)
  fir_col_async4/61(real_back_out15) -> fir_col_async3/61(real_back15)
  fir_col_async4/62(imag_back_out15) -> fir_col_async3/62(imag_back15)
  fir_col_async4/63(real_back_out16) -> fir_col_async3/63(real_back16)
  fir_col_async4/64(imag_back_out16) -> fir_col_async3/64(imag_back16)
  fir_col_async5/33(real_back_out1) -> fir_col_async4/33(real_back1)
  fir_col_async5/34(imag_back_out1) -> fir_col_async4/34(imag_back1)
  fir_col_async5/35(real_back_out2) -> fir_col_async4/35(real_back2)
  fir_col_async5/36(imag_back_out2) -> fir_col_async4/36(imag_back2)
  fir_col_async5/37(real_back_out3) -> fir_col_async4/37(real_back3)
  fir_col_async5/38(imag_back_out3) -> fir_col_async4/38(imag_back3)
  fir_col_async5/39(real_back_out4) -> fir_col_async4/39(real_back4)
  fir_col_async5/40(imag_back_out4) -> fir_col_async4/40(imag_back4)
  fir_col_async5/41(real_back_out5) -> fir_col_async4/41(real_back5)
  fir_col_async5/42(imag_back_out5) -> fir_col_async4/42(imag_back5)
  fir_col_async5/43(real_back_out6) -> fir_col_async4/43(real_back6)
  fir_col_async5/44(imag_back_out6) -> fir_col_async4/44(imag_back6)
  fir_col_async5/45(real_back_out7) -> fir_col_async4/45(real_back7)
  fir_col_async5/46(imag_back_out7) -> fir_col_async4/46(imag_back7)
  fir_col_async5/47(real_back_out8) -> fir_col_async4/47(real_back8)
  fir_col_async5/48(imag_back_out8) -> fir_col_async4/48(imag_back8)
  fir_col_async5/49(real_back_out9) -> fir_col_async4/49(real_back9)
  fir_col_async5/50(imag_back_out9) -> fir_col_async4/50(imag_back9)
  fir_col_async5/51(real_back_out10) -> fir_col_async4/51(real_back10)
  fir_col_async5/52(imag_back_out10) -> fir_col_async4/52(imag_back10)
  fir_col_async5/53(real_back_out11) -> fir_col_async4/53(real_back11)
  fir_col_async5/54(imag_back_out11) -> fir_col_async4/54(imag_back11)
  fir_col_async5/55(real_back_out12) -> fir_col_async4/55(real_back12)
  fir_col_async5/56(imag_back_out12) -> fir_col_async4/56(imag_back12)
  fir_col_async5/57(real_back_out13) -> fir_col_async4/57(real_back13)
  fir_col_async5/58(imag_back_out13) -> fir_col_async4/58(imag_back13)
  fir_col_async5/59(real_back_out14) -> fir_col_async4/59(real_back14)
  fir_col_async5/60(imag_back_out14) -> fir_col_async4/60(imag_back14)
  fir_col_async5/61(real_back_out15) -> fir_col_async4/61(real_back15)
  fir_col_async5/62(imag_back_out15) -> fir_col_async4/62(imag_back15)
  fir_col_async5/63(real_back_out16) -> fir_col_async4/63(real_back16)
  fir_col_async5/64(imag_back_out16) -> fir_col_async4/64(imag_back16)
  fir_col_async6/33(real_back_out1) -> fir_col_async5/33(real_back1)
  fir_col_async6/34(imag_back_out1) -> fir_col_async5/34(imag_back1)
  fir_col_async6/35(real_back_out2) -> fir_col_async5/35(real_back2)
  fir_col_async6/36(imag_back_out2) -> fir_col_async5/36(imag_back2)
  fir_col_async6/37(real_back_out3) -> fir_col_async5/37(real_back3)
  fir_col_async6/38(imag_back_out3) -> fir_col_async5/38(imag_back3)
  fir_col_async6/39(real_back_out4) -> fir_col_async5/39(real_back4)
  fir_col_async6/40(imag_back_out4) -> fir_col_async5/40(imag_back4)
  fir_col_async6/41(real_back_out5) -> fir_col_async5/41(real_back5)
  fir_col_async6/42(imag_back_out5) -> fir_col_async5/42(imag_back5)
  fir_col_async6/43(real_back_out6) -> fir_col_async5/43(real_back6)
  fir_col_async6/44(imag_back_out6) -> fir_col_async5/44(imag_back6)
  fir_col_async6/45(real_back_out7) -> fir_col_async5/45(real_back7)
  fir_col_async6/46(imag_back_out7) -> fir_col_async5/46(imag_back7)
  fir_col_async6/47(real_back_out8) -> fir_col_async5/47(real_back8)
  fir_col_async6/48(imag_back_out8) -> fir_col_async5/48(imag_back8)
  fir_col_async6/49(real_back_out9) -> fir_col_async5/49(real_back9)
  fir_col_async6/50(imag_back_out9) -> fir_col_async5/50(imag_back9)
  fir_col_async6/51(real_back_out10) -> fir_col_async5/51(real_back10)
  fir_col_async6/52(imag_back_out10) -> fir_col_async5/52(imag_back10)
  fir_col_async6/53(real_back_out11) -> fir_col_async5/53(real_back11)
  fir_col_async6/54(imag_back_out11) -> fir_col_async5/54(imag_back11)
  fir_col_async6/55(real_back_out12) -> fir_col_async5/55(real_back12)
  fir_col_async6/56(imag_back_out12) -> fir_col_async5/56(imag_back12)
  fir_col_async6/57(real_back_out13) -> fir_col_async5/57(real_back13)
  fir_col_async6/58(imag_back_out13) -> fir_col_async5/58(imag_back13)
  fir_col_async6/59(real_back_out14) -> fir_col_async5/59(real_back14)
  fir_col_async6/60(imag_back_out14) -> fir_col_async5/60(imag_back14)
  fir_col_async6/61(real_back_out15) -> fir_col_async5/61(real_back15)
  fir_col_async6/62(imag_back_out15) -> fir_col_async5/62(imag_back15)
  fir_col_async6/63(real_back_out16) -> fir_col_async5/63(real_back16)
  fir_col_async6/64(imag_back_out16) -> fir_col_async5/64(imag_back16)
  fir_col_async7/33(real_back_out1) -> fir_col_async6/33(real_back1)
  fir_col_async7/34(imag_back_out1) -> fir_col_async6/34(imag_back1)
  fir_col_async7/35(real_back_out2) -> fir_col_async6/35(real_back2)
  fir_col_async7/36(imag_back_out2) -> fir_col_async6/36(imag_back2)
  fir_col_async7/37(real_back_out3) -> fir_col_async6/37(real_back3)
  fir_col_async7/38(imag_back_out3) -> fir_col_async6/38(imag_back3)
  fir_col_async7/39(real_back_out4) -> fir_col_async6/39(real_back4)
  fir_col_async7/40(imag_back_out4) -> fir_col_async6/40(imag_back4)
  fir_col_async7/41(real_back_out5) -> fir_col_async6/41(real_back5)
  fir_col_async7/42(imag_back_out5) -> fir_col_async6/42(imag_back5)
  fir_col_async7/43(real_back_out6) -> fir_col_async6/43(real_back6)
  fir_col_async7/44(imag_back_out6) -> fir_col_async6/44(imag_back6)
  fir_col_async7/45(real_back_out7) -> fir_col_async6/45(real_back7)
  fir_col_async7/46(imag_back_out7) -> fir_col_async6/46(imag_back7)
  fir_col_async7/47(real_back_out8) -> fir_col_async6/47(real_back8)
  fir_col_async7/48(imag_back_out8) -> fir_col_async6/48(imag_back8)
  fir_col_async7/49(real_back_out9) -> fir_col_async6/49(real_back9)
  fir_col_async7/50(imag_back_out9) -> fir_col_async6/50(imag_back9)
  fir_col_async7/51(real_back_out10) -> fir_col_async6/51(real_back10)
  fir_col_async7/52(imag_back_out10) -> fir_col_async6/52(imag_back10)
  fir_col_async7/53(real_back_out11) -> fir_col_async6/53(real_back11)
  fir_col_async7/54(imag_back_out11) -> fir_col_async6/54(imag_back11)
  fir_col_async7/55(real_back_out12) -> fir_col_async6/55(real_back12)
  fir_col_async7/56(imag_back_out12) -> fir_col_async6/56(imag_back12)
  fir_col_async7/57(real_back_out13) -> fir_col_async6/57(real_back13)
  fir_col_async7/58(imag_back_out13) -> fir_col_async6/58(imag_back13)
  fir_col_async7/59(real_back_out14) -> fir_col_async6/59(real_back14)
  fir_col_async7/60(imag_back_out14) -> fir_col_async6/60(imag_back14)
  fir_col_async7/61(real_back_out15) -> fir_col_async6/61(real_back15)
  fir_col_async7/62(imag_back_out15) -> fir_col_async6/62(imag_back15)
  fir_col_async7/63(real_back_out16) -> fir_col_async6/63(real_back16)
  fir_col_async7/64(imag_back_out16) -> fir_col_async6/64(imag_back16)
  fir_col_async8/33(real_back_out1) -> fir_col_async7/33(real_back1)
  fir_col_async8/34(imag_back_out1) -> fir_col_async7/34(imag_back1)
  fir_col_async8/35(real_back_out2) -> fir_col_async7/35(real_back2)
  fir_col_async8/36(imag_back_out2) -> fir_col_async7/36(imag_back2)
  fir_col_async8/37(real_back_out3) -> fir_col_async7/37(real_back3)
  fir_col_async8/38(imag_back_out3) -> fir_col_async7/38(imag_back3)
  fir_col_async8/39(real_back_out4) -> fir_col_async7/39(real_back4)
  fir_col_async8/40(imag_back_out4) -> fir_col_async7/40(imag_back4)
  fir_col_async8/41(real_back_out5) -> fir_col_async7/41(real_back5)
  fir_col_async8/42(imag_back_out5) -> fir_col_async7/42(imag_back5)
  fir_col_async8/43(real_back_out6) -> fir_col_async7/43(real_back6)
  fir_col_async8/44(imag_back_out6) -> fir_col_async7/44(imag_back6)
  fir_col_async8/45(real_back_out7) -> fir_col_async7/45(real_back7)
  fir_col_async8/46(imag_back_out7) -> fir_col_async7/46(imag_back7)
  fir_col_async8/47(real_back_out8) -> fir_col_async7/47(real_back8)
  fir_col_async8/48(imag_back_out8) -> fir_col_async7/48(imag_back8)
  fir_col_async8/49(real_back_out9) -> fir_col_async7/49(real_back9)
  fir_col_async8/50(imag_back_out9) -> fir_col_async7/50(imag_back9)
  fir_col_async8/51(real_back_out10) -> fir_col_async7/51(real_back10)
  fir_col_async8/52(imag_back_out10) -> fir_col_async7/52(imag_back10)
  fir_col_async8/53(real_back_out11) -> fir_col_async7/53(real_back11)
  fir_col_async8/54(imag_back_out11) -> fir_col_async7/54(imag_back11)
  fir_col_async8/55(real_back_out12) -> fir_col_async7/55(real_back12)
  fir_col_async8/56(imag_back_out12) -> fir_col_async7/56(imag_back12)
  fir_col_async8/57(real_back_out13) -> fir_col_async7/57(real_back13)
  fir_col_async8/58(imag_back_out13) -> fir_col_async7/58(imag_back13)
  fir_col_async8/59(real_back_out14) -> fir_col_async7/59(real_back14)
  fir_col_async8/60(imag_back_out14) -> fir_col_async7/60(imag_back14)
  fir_col_async8/61(real_back_out15) -> fir_col_async7/61(real_back15)
  fir_col_async8/62(imag_back_out15) -> fir_col_async7/62(imag_back15)
  fir_col_async8/63(real_back_out16) -> fir_col_async7/63(real_back16)
  fir_col_async8/64(imag_back_out16) -> fir_col_async7/64(imag_back16)
  fir_col_async8/1(real_out1) -> fir_col_async8/33(real_back1)
  fir_col_async8/2(imag_out1) -> fir_col_async8/34(imag_back1)
  fir_col_async8/3(real_out2) -> fir_col_async8/35(real_back2)
  fir_col_async8/4(imag_out2) -> fir_col_async8/36(imag_back2)
  fir_col_async8/5(real_out3) -> fir_col_async8/37(real_back3)
  fir_col_async8/6(imag_out3) -> fir_col_async8/38(imag_back3)
  fir_col_async8/7(real_out4) -> fir_col_async8/39(real_back4)
  fir_col_async8/8(imag_out4) -> fir_col_async8/40(imag_back4)
  fir_col_async8/9(real_out5) -> fir_col_async8/41(real_back5)
  fir_col_async8/10(imag_out5) -> fir_col_async8/42(imag_back5)
  fir_col_async8/11(real_out6) -> fir_col_async8/43(real_back6)
  fir_col_async8/12(imag_out6) -> fir_col_async8/44(imag_back6)
  fir_col_async8/13(real_out7) -> fir_col_async8/45(real_back7)
  fir_col_async8/14(imag_out7) -> fir_col_async8/46(imag_back7)
  fir_col_async8/15(real_out8) -> fir_col_async8/47(real_back8)
  fir_col_async8/16(imag_out8) -> fir_col_async8/48(imag_back8)
  fir_col_async8/17(real_out9) -> fir_col_async8/49(real_back9)
  fir_col_async8/18(imag_out9) -> fir_col_async8/50(imag_back9)
  fir_col_async8/19(real_out10) -> fir_col_async8/51(real_back10)
  fir_col_async8/20(imag_out10) -> fir_col_async8/52(imag_back10)
  fir_col_async8/21(real_out11) -> fir_col_async8/53(real_back11)
  fir_col_async8/22(imag_out11) -> fir_col_async8/54(imag_back11)
  fir_col_async8/23(real_out12) -> fir_col_async8/55(real_back12)
  fir_col_async8/24(imag_out12) -> fir_col_async8/56(imag_back12)
  fir_col_async8/25(real_out13) -> fir_col_async8/57(real_back13)
  fir_col_async8/26(imag_out13) -> fir_col_async8/58(imag_back13)
  fir_col_async8/27(real_out14) -> fir_col_async8/59(real_back14)
  fir_col_async8/28(imag_out14) -> fir_col_async8/60(imag_back14)
  fir_col_async8/29(real_out15) -> fir_col_async8/61(real_back15)
  fir_col_async8/30(imag_out15) -> fir_col_async8/62(imag_back15)
  fir_col_async8/31(real_out16) -> fir_col_async8/63(real_back16)
  fir_col_async8/32(imag_out16) -> fir_col_async8/64(imag_back16)
